simulink model "Inverter_pq_comp"  (R2023b)
settings: Solver=FixedStepDiscrete  StartTime=0.0  StopTime=0.04  RelTol=1e-3  EnableMultiTasking=on
InitFcn:
  | %% Definition of the parameters
  | 
  | Parameter_Definition
  | 
  | %% Damping
  | 
  | Rd = 3.9;
  | 
  | %% PRes Gains Calculation
  | 
  | % Definicao das grandezas
  | w_cl = 1j*2*pi*1200;  % Phase Crossing Frequency
  | no   = 1;           % Integral Resonant Constant
  | A    = 1;             % Carrier Amplitude
  | 
  | % Kp calculation
  | a0 = 1;
  | a1 = Rd*Cf;
  | b0 = 0;
  | b1 = Lf+Lg;
  | b2 = Rd*Lf*Cf+Rd*Lg*Cf;
  | b3 = Lf*Lg*Cf;
  | 
  | G_lcl = (a1*w_cl+a0)/(b3*w_cl^3+b2*w_cl^2+b1*w_cl+b0);
  | % G_lcl = 1/((Lf+Lg)*w_cl+Rf);
  | 
  | G_PWM = (1/A)*(1-w_cl*Ts/4)/(1+w_cl*Ts/4);
  | 
  | G_wc  = (Vdc/2)*(1/I_base)*G_lcl*G_PWM;
  | 
  | G_wc_abs = abs(G_wc);
  | 
  | Kp = 1/G_wc_abs;
  | 
  | % Discretized Controller Gains
  | ressonance_list = [1,5,7];
  | 
  | n_res = length(ressonance_list);
  | a = zeros(2,n_res);
  | b = zeros(2,n_res);
  | Ki_res = zeros(1,n_res);
  | 
  | % for i = 1:n_res
  | %   k = ressonance_list(i);
  | %   Ki_res(i) = (2.2*Kp)/(no*T_gr);
  | %   a(i) = (2*Ki_res(i)*Ts)/(4+((k*w_gr)^2)*Ts^2);
  | %   b(i) = (-8+2*((k*w_gr)^2)*Ts^2)/(4+((k*w_gr)^2)*Ts^2);
  | % end
  | 
  | % wc is the cutoff frequency/damping factor in rad/s
  | wc = 5;
  | 
  | for i = 1:n_res
  |   k = ressonance_list(i);
  |   wk = k * w_gr; % Resonant frequency for this harmonic
  | 
  |   Ki_res(i) = (2.2*Kp)/(0.8*no*T_gr);
  | 
  |   % 1. Calculate the common denominator
  |   den = 4 + 4*wc*Ts + (wk^2)*(Ts^2);
  | ... (+14 lines)
values from neighbouring files (symbols this model uses):
  a1_sogi = single(2*(w0_sogi^2-c_sogi^2)/den0_sogi)    [Parameter_Definition.m]
  a2_sogi = single((c_sogi^2                 - k_sogi*w0_sogi*c_sogi                 + w0_sogi^2)/den0_sogi)    [Parameter_Definition.m]
  bD_sogi = single(k_sogi*w0_sogi*c_sogi/den0_sogi)    [Parameter_Definition.m]
  bQ_sogi = single(k_sogi*w0_sogi^2/den0_sogi)    [Parameter_Definition.m]
  Cf = 5e-6    (= 5e-06)    [Parameter_Definition.m]
  I_base = S_base/(sqrt(3)*V_gr)    [Parameter_Definition.m]
  K_i = 1/25    (= 0.04)    [Parameter_Definition.m]
  K_vc = 1/200    (= 0.005)    [Parameter_Definition.m]
  K_vdc = 1/500    (= 0.002)    [Parameter_Definition.m]
  Lf = 1e-3    (= 0.001)    [Parameter_Definition.m]
  Lg = 0.5e-3    (= 0.0005)    [Parameter_Definition.m]
  S_base = S_rated    (= 1000)    [Parameter_Definition.m]
  Ts = 2*(4167)/100e6    (= 8.334e-05)    [Parameter_Definition.m]
  V_base = sqrt(3)*V_gr    [Parameter_Definition.m]
  Vdc = 800    [Parameter_Definition.m]
  Vdc_base = Vdc    (= 800)    [Parameter_Definition.m]
  w_gr = 2*pi*f_gr    (= 376.991118431)    [Parameter_Definition.m]
undefined symbols (not defined in the file or in its folder): Down, GPTRIP1SEL, TZ1, Up
libraries: c2802xlib x32, c2837xDlib x4, simulink x1
(part 2 of 2)

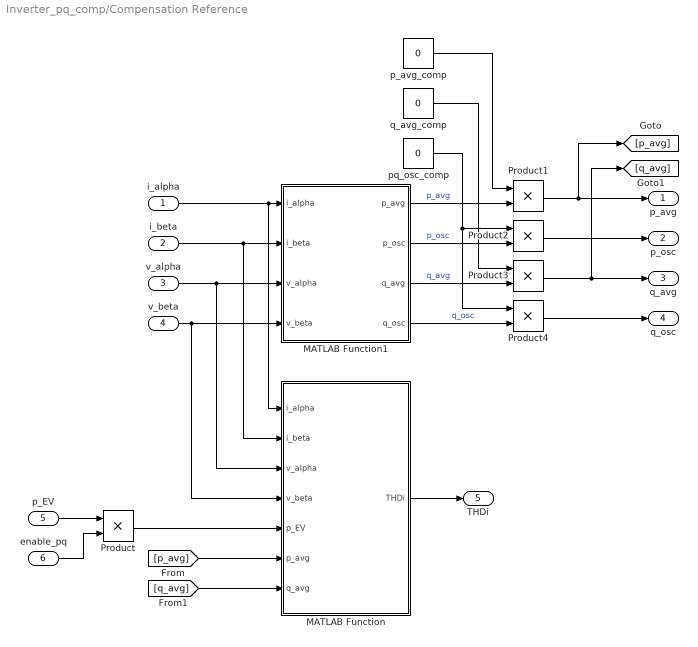
== system Inverter_pq_comp/Compensation Reference ==
  i_alpha : Inport
  i_beta : Inport  Port=2
  v_alpha : Inport  Port=3
  v_beta : Inport  Port=4
  p_EV : Inport  Port=5
  enable_pq : Inport  Port=6
  MATLAB Function : MATLAB Function  TreatAsAtomicUnit=on
  MATLAB Function1 : MATLAB Function  TreatAsAtomicUnit=on
  Product{,1..4} (5 alike) : Product
  p_avg_comp : Constant  Value=0  OutDataTypeStr=single
  pq_osc_comp : Constant  Value=0  OutDataTypeStr=single
  q_avg_comp : Constant  Value=0  OutDataTypeStr=single
  p_avg : Outport
  p_osc : Outport  Port=2
  q_avg : Outport  Port=3
  q_osc : Outport  Port=4
  THDi : Outport  Port=5
  wires:
  MATLAB Function1/1(p_avg) -> Product1/2  "p_avg"
  MATLAB Function1/3(q_avg) -> Product3/2  "q_avg"
  MATLAB Function1/2(p_osc) -> Product2/2  "p_osc"
  i_alpha/1 -> MATLAB Function/1(i_alpha), MATLAB Function1/1(i_alpha)
  MATLAB Function1/4(q_osc) -> Product4/2  "q_osc"
  i_beta/1 -> MATLAB Function/2(i_beta), MATLAB Function1/2(i_beta)
  v_alpha/1 -> MATLAB Function/3(v_alpha), MATLAB Function1/3(v_alpha)
  v_beta/1 -> MATLAB Function/4(v_beta), MATLAB Function1/4(v_beta)
  Product1/1 -> [p_avg], p_avg/1
  Product2/1 -> p_osc/1
  Product3/1 -> [q_avg], q_avg/1
  Product4/1 -> q_osc/1
  [p_avg] -> MATLAB Function/6(p_avg)
  [q_avg] -> MATLAB Function/7(q_avg)
  MATLAB Function/1(THDi) -> THDi/1
  Product/1 -> MATLAB Function/5(p_EV)
  p_EV/1 -> Product/1
  enable_pq/1 -> Product/2
  p_avg_comp/1 -> Product1/1
  q_avg_comp/1 -> Product3/1
  pq_osc_comp/1 -> Product4/1, Product2/1

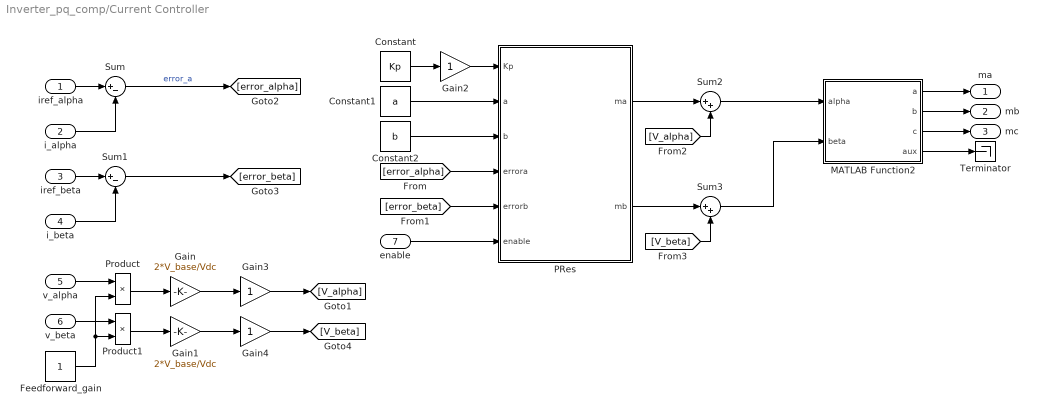
== system Inverter_pq_comp/Current Controller ==
  iref_alpha : Inport
  i_alpha : Inport  Port=2
  iref_beta : Inport  Port=3
  i_beta : Inport  Port=4
  v_alpha : Inport  Port=5
  v_beta : Inport  Port=6
  enable : Inport  Port=7
  Constant : Constant  Value=Kp  OutDataTypeStr=single
  Constant1 : Constant  Value=a  OutDataTypeStr=single
  Constant2 : Constant  Value=b  OutDataTypeStr=single
  Feedforward_gain : Constant  OutDataTypeStr=single
  Gain : Gain  Gain=2*V_base/Vdc
  Gain1 : Gain  Gain=2*V_base/Vdc
  Gain2 : Gain
  Gain3 : Gain
  Gain4 : Gain
  MATLAB Function2 : MATLAB Function  TreatAsAtomicUnit=on
  PRes : MATLAB Function  TreatAsAtomicUnit=on
  Product : Product
  Product1 : Product
  Sum : Sum  Inputs=|+-
  Sum1 : Sum  Inputs=|+-
  Sum2 : Sum  Inputs=|++
  Sum3 : Sum  Inputs=|++
  Terminator : Terminator
  ma : Outport
  mb : Outport  Port=2
  mc : Outport  Port=3
  wires:
  Constant1/1 -> PRes/2(a)
  Constant2/1 -> PRes/3(b)
  [error_alpha] -> PRes/4(errora)
  [error_beta] -> PRes/5(errorb)
  iref_alpha/1 -> Sum/1
  i_alpha/1 -> Sum/2
  iref_beta/1 -> Sum1/1
  i_beta/1 -> Sum1/2
  Sum1/1 -> [error_beta]
  Sum/1 -> [error_alpha]  "error_a"
  enable/1 -> PRes/6(enable)
  PRes/1(ma) -> Sum2/1
  Sum2/1 -> MATLAB Function2/1(alpha)
  PRes/2(mb) -> Sum3/1
  [V_alpha] -> Sum2/2
  [V_beta] -> Sum3/2
  v_beta/1 -> Product1/1
  Product1/1 -> Gain1/1
  v_alpha/1 -> Product/1
  Product/1 -> Gain/1
  Feedforward_gain/1 -> Product/2, Product1/2
  Constant/1 -> Gain2/1
  MATLAB Function2/1(a) -> ma/1
  MATLAB Function2/2(b) -> mb/1
  MATLAB Function2/3(c) -> mc/1
  MATLAB Function2/4(aux) -> Terminator/1
  Sum3/1 -> MATLAB Function2/2(beta)
  Gain/1 -> Gain3/1
  Gain1/1 -> Gain4/1
  Gain2/1 -> PRes/1(Kp)
  Gain3/1 -> [V_alpha]
  Gain4/1 -> [V_beta]

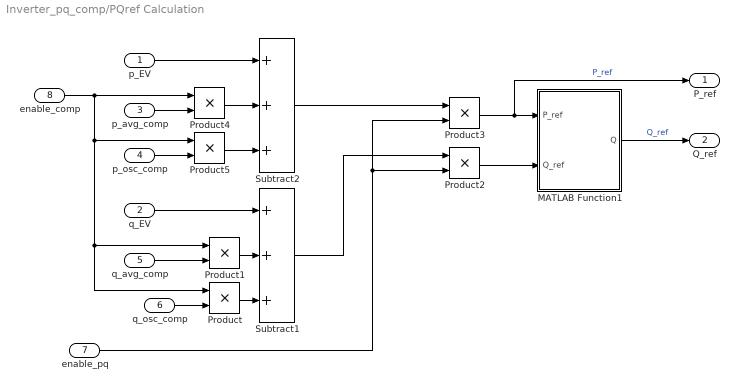
== system Inverter_pq_comp/PQref Calculation ==
  p_EV : Inport
  q_EV : Inport  Port=2
  p_avg_comp : Inport  Port=3
  p_osc_comp : Inport  Port=4
  q_avg_comp : Inport  Port=5
  q_osc_comp : Inport  Port=6
  enable_pq : Inport  Port=7
  enable_comp : Inport  Port=8
  MATLAB Function1 : MATLAB Function  TreatAsAtomicUnit=on
  Product{,1..5} (6 alike) : Product
  Subtract1 : Sum  Inputs=+++
  Subtract2 : Sum  Inputs=+++
  P_ref : Outport
  Q_ref : Outport  Port=2
  wires:
  p_osc_comp/1 -> Product5/2
  Product/1 -> Subtract1/3
  MATLAB Function1/1(Q) -> Q_ref/1  "Q_ref"
  Product1/1 -> Subtract1/2
  p_avg_comp/1 -> Product4/2
  q_osc_comp/1 -> Product/2
  q_avg_comp/1 -> Product1/2
  Product4/1 -> Subtract2/2
  p_EV/1 -> Subtract2/1
  Product5/1 -> Subtract2/3
  q_EV/1 -> Subtract1/1
  Subtract1/1 -> Product2/1
  Product2/1 -> MATLAB Function1/2(Q_ref)
  Product3/1 -> P_ref/1, MATLAB Function1/1(P_ref)  "P_ref"
  enable_pq/1 -> Product3/2, Product2/2
  Subtract2/1 -> Product3/1
  enable_comp/1 -> Product/1, Product1/1, Product5/1, Product4/1

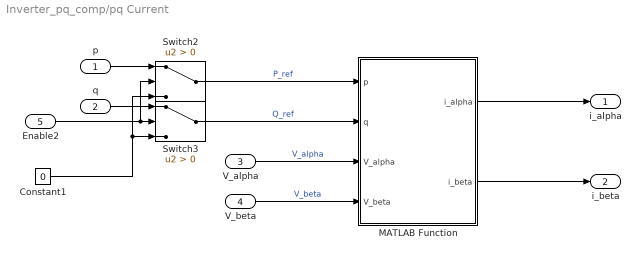
== system Inverter_pq_comp/pq Current ==
  p : Inport
  q : Inport  Port=2
  V_alpha : Inport  Port=3
  V_beta : Inport  Port=4
  Enable2 : Inport  Port=5
  Constant1 : Constant  Value=0  OutDataTypeStr=single
  MATLAB Function : MATLAB Function  TreatAsAtomicUnit=on
  Switch2 : Switch  Criteria=u2 > Threshold  SaturateOnIntegerOverflow=off  InputSameDT=off
  Switch3 : Switch  Criteria=u2 > Threshold  SaturateOnIntegerOverflow=off  InputSameDT=off
  i_alpha : Outport
  i_beta : Outport  Port=2
  wires:
  V_beta/1 -> MATLAB Function/4(V_beta)  "V_beta"
  V_alpha/1 -> MATLAB Function/3(V_alpha)  "V_alpha"
  MATLAB Function/1(i_alpha) -> i_alpha/1
  MATLAB Function/2(i_beta) -> i_beta/1
  p/1 -> Switch2/1
  Switch3/1 -> MATLAB Function/2(q)  "Q_ref"
  q/1 -> Switch3/1
  Constant1/1 -> Switch2/3, Switch3/3
  Enable2/1 -> Switch2/2, Switch3/2
  Switch2/1 -> MATLAB Function/1(p)  "P_ref"

== matlab function Inverter_pq_comp/RMS_fcn4 ==
  data: RMSin input; yout output
function yout = fcn(RMSin)

win = 200;

persistent sampleRMS
    if isempty(sampleRMS)
        sampleRMS = single(0.0);
    end
    if sampleRMS>=win
        sampleRMS = single(0.0);
    end

persistent RMSout
if isempty(RMSout)
    RMSout = single(0.0);
end    
persistent sumRMS
if isempty(sumRMS)
    sumRMS = single(0.0);
end
persistent RMSinArray
     if isempty(RMSinArray)
         RMSinArray = zeros(1,win);
     end

sampleRMS = sampleRMS + 1;      

%RMS of Input Signal
sumRMS = sumRMS + RMSin*RMSin - RMSinArray(1,sampleRMS);
RMSinArray(1,sampleRMS) = RMSin*RMSin;
if sumRMS>=0.0
    RMSout = sqrt(sumRMS/win);
end

%RMSout = RMSout_temp;

yout = RMSout;

== matlab function Inverter_pq_comp/RMS_fcn5 ==
  data: RMSin input; yout output
function yout = fcn(RMSin)

win = 200;

persistent sampleRMS
    if isempty(sampleRMS)
        sampleRMS = single(0.0);
    end
    if sampleRMS>=win
        sampleRMS = single(0.0);
    end

persistent RMSout
if isempty(RMSout)
    RMSout = single(0.0);
end    
persistent sumRMS
if isempty(sumRMS)
    sumRMS = single(0.0);
end
persistent RMSinArray
     if isempty(RMSinArray)
         RMSinArray = zeros(1,win);
     end

sampleRMS = sampleRMS + 1;      

%RMS of Input Signal
sumRMS = sumRMS + RMSin*RMSin - RMSinArray(1,sampleRMS);
RMSinArray(1,sampleRMS) = RMSin*RMSin;
if sumRMS>=0.0
    RMSout = sqrt(sumRMS/win);
end

%RMSout = RMSout_temp;

yout = RMSout;

== matlab function Inverter_pq_comp/Compensation Reference/MATLAB Function1 ==
  data: i_alpha input; p_avg output; i_beta input; v_alpha input; v_beta input; p_osc output; q_avg output; q_osc output
function [p_avg, p_osc, q_avg, q_osc] = pqCalc(i_alpha, i_beta, v_alpha, v_beta)
    % Initial logic and parameters are validated. 
    % Standard processing applied for spatial vector alignment.

    persistent buffer_p buffer_q sum_p sum_q idx
    window = 200; % Must match your 12000Hz/60Hz window size exactly
    
    if isempty(buffer_p)
        buffer_p = zeros(window, 1);
        buffer_q = zeros(window, 1);
        sum_p = single(0.0);
        sum_q = single(0.0);
        idx = 1;
    end
    
    % Final transformation: Strip scaling coefficients to match I_total_sq domain
    p = (v_alpha * i_alpha) + (v_beta * i_beta);
    q = (v_beta * i_alpha) - (v_alpha * i_beta);
    
    % Align filter topology to match current/voltage sliding window
    old_p = buffer_p(idx);
    old_q = buffer_q(idx);
    
    buffer_p(idx) = p;
    buffer_q(idx) = q;
    
    sum_p = sum_p + p - old_p;
    sum_q = sum_q + q - old_q;
    
    idx = idx + 1;
    if idx > window
        idx = 1;
    end
    
    p_avg = sum_p / window;
    q_avg = sum_q / window;
    
    p_osc = p - p_avg;
    q_osc = q - q_avg;
end

== matlab function Inverter_pq_comp/MATLAB Function11 ==
  data: i_rms input; error_overcurrent output; error_ac_overvoltage output; error_dc_overvoltage output; error_unbalance output; error_low_Vdc output; enable_contactor_out output; enable_PreCharge_out output; enable_PWM_out output; enable_PQ_out output; enable_comp_out output; enable_Feedforward_out output; I_limit input; V_rms input; V_limit input; V_dc input; Vdc_limit input; V_unb input; Vunb_limit input; enable_relay input; enable_PWM input; enable_PreCharge input; enable_PQ input; enable_comp input; error_reset input; error_reset_out output; out_gpio output
function [error_overcurrent, error_ac_overvoltage, error_dc_overvoltage, error_unbalance, error_low_Vdc, enable_contactor_out, enable_PreCharge_out, enable_PWM_out, enable_PQ_out, enable_comp_out, enable_Feedforward_out, error_reset_out, out_gpio] = TNPC_Protection(i_rms, I_limit, V_rms, V_limit, V_dc, Vdc_limit, V_unb, Vunb_limit, enable_relay, enable_PWM, enable_PreCharge, enable_PQ, enable_comp, error_reset)

% Persistent variables definition
persistent error_flag
persistent error_overcurrent_p
persistent error_ac_overvoltage_p
persistent error_dc_overvoltage_p
persistent error_unbalance_p
persistent error_low_Vdc_p
persistent count_I_limit
if isempty(error_flag)
    error_flag = single(0);
    error_overcurrent_p    = single(0);
    error_ac_overvoltage_p = single(0);
    error_dc_overvoltage_p = single(0);
    error_unbalance_p      = single(0);
    error_low_Vdc_p        = single(0);
    count_I_limit          = int16(0);
end


out_Feedforward = single(0.0);
% Count to keep high current limit in first 15 cycles
if enable_relay == 1
    if count_I_limit < 10*200
        I_limit = single(100.0);
        count_I_limit = count_I_limit + 1;
        out_Feedforward = single(1.0);
    elseif count_I_limit < 15*200
        I_limit = single(100.0);
        count_I_limit = count_I_limit + 1;
        out_Feedforward = single(0.0);
    end
end

enable_Feedforward_out = out_Feedforward;

% Check for errors
if max(i_rms) > I_limit
    error_overcurrent = single(1);
    error_overcurrent_p = single(1);
else
    error_overcurrent = single(0);
end

if V_dc > Vdc_limit
    error_dc_overvoltage = single(1);
    error_dc_overvoltage_p = single(1);
else
    error_dc_overvoltage = single(0);  
end

if V_unb > Vunb_limit
    error_unbalance = single(1);
    error_unbalance_p = single(1);
else
    error_unbalance = single(0);
end

if max(V_rms) > V_limit
    error_ac_overvoltage = single(1);
    error_ac_overvoltage_p = single(1);
else
    error_ac_overvoltage = single(0);  
end

if V_dc*500 < sqrt(2)*max(V_rms)*250
    error_low_Vdc = single(1);
    error_low_Vdc_p = single(1);
else
    error_low_Vdc = single(0);
end

% Raise the error flag
if (error_overcurrent == 1) || (error_dc_overvoltage == 1) || (error_unbalance == 1) || (error_ac_overvoltage == 1) || (error_low_Vdc == 1)
    error_flag = single(1);
end

% Reset logic
if error_flag == 1 && error_reset == 1 && error_overcurrent == 0 && error_dc_overvoltage == 0 && error_ac_overvoltage == 0 && error_unbalance == 0 && error_low_Vdc == 0
    % Clear the persistent variables
    error_flag = single(0);
    error_overcurrent_p    = single(0);
    error_ac_overvoltage_p = single(0);
    error_dc_overvoltage_p = single(0);
    error_unbalance_p      = single(0);
    error_low_Vdc_p        = single(0);
    count_I_limit          = int16(0);
    % Send 0 to the reset signal
    error_reset_out = single(0);
else
    error_reset_out = error_reset;
end

% Enable signals output
if error_flag == 1
    enable_contactor_out = single(0);
    enable_PWM_out       = single(0);
    enable_PreCharge_out = single(0);
    enable_PQ_out        = single(0);
    enable_comp_out      = single(0);
else
    enable_contactor_out = enable_relay;
    enable_PWM_out       = enable_PWM;
    enable_PreCharge_out = enable_PreCharge;
    enable_PQ_out        = enable_PQ;
    enable_comp_out      = enable_comp;
end

if (error_overcurrent_p == 1) || (error_dc_overvoltage_p == 1) || (error_unbalance_p == 1) || (error_ac_overvoltage_p == 1) || (error_low_Vdc_p == 1)
    out_gpio = single(1);
else
    out_gpio = single(0);
end

== matlab function Inverter_pq_comp/PQref Calculation/MATLAB Function1 ==
  data: P_ref input; Q_ref input; Q output
function Q = Q_limit(P_ref, Q_ref)

Smax = single(1.0);

if P_ref > 1
    P_ref = single(1.0);
end

Qmax = sqrt(Smax^2-P_ref^2);

if Qmax > abs(Q_ref)
    Q = Q_ref;
else
    Q = Qmax*sign(Q_ref);
end

== matlab function Inverter_pq_comp/Current Controller/PRes ==
  data: Kp input; a input; b input; errora input; ma output; errorb input; mb output; enable input
function [ma, mb] = PResCurrent(Kp, a, b, errora, errorb, enable)

%Controller modeled in abc frame, considering p.u. values

%%% Variables Definition
%%%%#########################################################
%%%%######################################################### 

nRes = length(a);

max_pu = single(1.0);

%Proportional part variable
%Phase a
persistent pia
    if isempty(pia)
        pia = single(0.0);
    end
%Phase b    
persistent pib
    if isempty(pib)
        pib = single(0.0);
    end 
    
%Resonant parts variables
%Phase a
persistent presa
    if isempty(presa)
        presa = zeros(1,nRes);
    end
persistent presa_1d %1 sample delay
    if isempty(presa_1d)
        presa_1d = zeros(1,nRes);
    end    
persistent presa_2d %2 samples delay
    if isempty(presa_2d)
        presa_2d = zeros(1,nRes);
    end
persistent presOUT_ia
    if isempty(presOUT_ia)
        presOUT_ia = single(0.0);
    end
    
%Phase b
persistent presb
    if isempty(presb)
        presb = zeros(1,nRes);
    end
persistent presb_1d %1 sample delay
    if isempty(presb_1d)
        presb_1d = zeros(1,nRes);
    end    
persistent presb_2d %2 samples delay
    if isempty(presb_2d)
        presb_2d = zeros(1,nRes);
    end
persistent presOUT_ib
    if isempty(presOUT_ib)
        presOUT_ib = single(0.0);
    end

%Error variables
%Phase a
% persistent errora %Actual error
%     if isempty(errora)
%         errora = 0.0;
%     end
persistent errora_0d %Actual error to delay
    if isempty(errora_0d)
        errora_0d = single(0.0);
    end
persistent errora_1d %1 sample delay
    if isempty(errora_1d)
        errora_1d = single(0.0);
    end    
persistent errora_2d %2 sample delay
    if isempty(errora_2d)
        errora_2d = single(0.0);
    end   
%Phase b
% persistent errorb %Actual error
%     if isempty(errorb)
%         errorb = 0.0;
%     end
persistent errorb_0d %Actual error to delay
    if isempty(errorb_0d)
        errorb_0d = single(0.0);
    end
persistent errorb_1d %1 sample delay
    if isempty(errorb_1d)
        errorb_1d = single(0.0);
    end    
persistent errorb_2d %2 sample delay
    if isempty(errorb_2d)
        errorb_2d = single(0.0);
    end

%%% Enable logic
%%%%#########################################################
%%%%#########################################################

if ~enable 
    % Define safe outputs
    ma = single(0.0);
    mb = single(0.0);
    mc = single(0.0);
    
    % Reset history registers for bumpless transfer
    pia = single(0.0); pib = single(0.0);
    
    presa       = zeros(1,nRes);
    presa_1d    = zeros(1,nRes);
    presa_2d    = zeros(1,nRes);
    presOUT_ia  = single(0.0);
    
    presb       = zeros(1,nRes);
    presb_1d    = zeros(1,nRes);
    presb_2d    = zeros(1,nRes);
    presOUT_ib  = single(0.0);
    
    errora_0d = single(0.0); errora_1d = single(0.0); errora_2d = single(0.0);
    errorb_0d = single(0.0); errorb_1d = single(0.0); errorb_2d = single(0.0);
    
    % Exit the function completely
    return; 
end

%%% PRes Current Controllers
%%%%#########################################################
%%%%#########################################################

%Proportional part
pia = errora*Kp;
pib = errorb*Kp;
    
    %Saturation - a
    if pia > max_pu 
        pia = max_pu;
    end
    if pia < -1*max_pu
        pia = -1*max_pu;
    end
    %Saturation - b
    if pib > max_pu
        pib = max_pu;
    end
    if pib < -1*max_pu
        pib = -1*max_pu;
    end   
    
    % %Anti-windup - a
    % if pia > 0.0
    %     limit_ia = max_pu - pia;
    % else
    %     limit_ia = 1 + pia;
    % end
    %  %Anti-windup - b
    % if pib > 0.0
    %     limit_ib = max_pu - pib;
    % else
    %     limit_ib = 1 + pib;
    % end
%     %Anti-windup - c
%     if pic > 0.0
%         limit_ic = max_pu - pic;
%     else
%         limit_ic = 1 + pic;
%     end    
    
    
%Resonant part
errora_2d = errora_1d;
errora_1d = errora_0d;
errora_0d = errora;

errorb_2d = errorb_1d;
errorb_1d = errorb_0d;
errorb_0d = errorb;
        
for i=1:nRes

    %leg a
    presa_2d(i) = presa_1d(i);
	presa_1d(i) = presa(i);
	presa(i) = a(1,i)*errora + a(2,i)*errora_2d - b(1,i)*presa_1d(i) - b(2,i)*presa_2d(i);    
    % if presa(i) > limit_ia
    %     presa(i) = limit_ia;
    % end
    % if presa(i) < -1*limit_ia
    %     presa(i) = -1*limit_ia;
    % end
 
    %leg b
    presb_2d(i) = presb_1d(i);
	presb_1d(i) = presb(i);
	presb(i) = a(1,i)*errorb + a(2,i)*errorb_2d - b(1,i)*presb_1d(i) - b(2,i)*presb_2d(i);    
    % if presb(i) > limit_ib
    %     presb(i) = limit_ib;
    % end
    % if presb(i) < -1*limit_ib
    %     presb(i) = -1*limit_ib;
    % end  
    
end

presOUT_ia = pia;
presOUT_ib = pib;

for i=1:nRes
    presOUT_ia = presOUT_ia + presa(i);
    presOUT_ib = presOUT_ib + presb(i);  
end

%Output for PWM
ma = presOUT_ia;
        %Saturation - ta
        if ma > max_pu 
            ma = max_pu;
        end
        if ma < -1*max_pu
            ma = -1*max_pu;
        end

mb = presOUT_ib;
        %Saturation - tb
        if mb > max_pu 
            mb = max_pu;
        end
        if mb < -1*max_pu
            mb = -1*max_pu;
        end
        
end

== matlab function Inverter_pq_comp/Current Controller/MATLAB Function2 ==
  data: alpha input; a output; beta input; b output; c output; aux output
function [a, b, c, aux] = abc(alpha, beta)

a = sqrt(2/3)*alpha;
b = sqrt(2/3)*(-1*alpha/2 + sqrt(3)*beta/2);
c = sqrt(2/3)*(-1*alpha/2 - sqrt(3)*beta/2);

max_mod = max(abs([a, b, c]));

if max_mod > 1
    scale = 1/max_mod;

    a = a*scale;
    b = b*scale;
    c = c*scale;

    aux = single(1.0);
else
    aux = single(0.0);
end

== matlab function Inverter_pq_comp/MATLAB Function3 ==
  data: a input; alpha output; b input; c input; beta output
function [alpha, beta] = alpha_beta(a, b, c)

alpha = sqrt(2/3)*(a - b/2 - c/2);
beta  = sqrt(2/3)*(sqrt(3)*b/2 - sqrt(3)*c/2);

== matlab function Inverter_pq_comp/pq Current/MATLAB Function ==
  data: p input; i_alpha output; q input; i_beta output; V_alpha input; V_beta input
function [i_alpha, i_beta] = pq_to_i(p, q, V_alpha, V_beta)

i_alpha = (1/(V_alpha^2+V_beta^2))*(V_alpha*p + V_beta*q);
i_beta  = (1/(V_alpha^2+V_beta^2))*(V_beta*p - V_alpha*q);

== matlab function Inverter_pq_comp/Compensation Reference/MATLAB Function ==
  data: i_alpha input; THDi output; i_beta input; v_alpha input; v_beta input; p_EV input; p_avg input; q_avg input
function THDi = THD_calc( ...
    i_alpha, i_beta, ...
    v_alpha, v_beta, ...
    p_EV, p_avg, q_avg)
%#codegen

    window = 200;
    epsilon = 1e-9;

    persistent buffer_I_total;
    persistent buffer_V;
    persistent sum_I_total;
    persistent sum_V;
    persistent idx;
    persistent count;

    if isempty(idx)
        buffer_I_total = zeros(window,1);
        buffer_V = zeros(window,1);

        sum_I_total = single(0.0);
        sum_V = single(0.0);

        idx = 1;
        count = 0;
    end

    % Load-current magnitude squared
    I_total_inst_sq = i_alpha^2 + i_beta^2;

    % Fundamental PCC-voltage magnitude squared
    V_inst_sq = v_alpha^2 + v_beta^2;

    % Remove oldest samples
    old_I = buffer_I_total(idx);
    old_V = buffer_V(idx);

    % Insert newest samples
    buffer_I_total(idx) = I_total_inst_sq;
    buffer_V(idx) = V_inst_sq;

    % Update moving sums
    sum_I_total = ...
        sum_I_total + I_total_inst_sq - old_I;

    sum_V = ...
        sum_V + V_inst_sq - old_V;

    idx = idx + 1;

    if idx > window
        idx = 1;
    end

    if count < window
        count = count + 1;
    end

    % Do not calculate THD before one complete cycle
    if count < window
        THDi = single(0.0);
        return;
    end

    % Squared total load-current magnitude
    IL_total_sq = max(sum_I_total/window,0);

    % Squared fundamental voltage magnitude
    V1_sq = max(sum_V/window,epsilon);

    % Fundamental LOAD current
    IL_fund_sq = ...
        (p_avg^2 + q_avg^2)/V1_sq;

    % Harmonic LOAD current
    IH_load_sq = max( ...
        IL_total_sq - IL_fund_sq, ...
        0);

    % Fundamental grid current including EV charging
    %
    % Current convention:
    % p_EV is negative during charging.
    p_total_fund = p_avg - p_EV;

    IT_fund_sq = ...
        (p_total_fund^2 + q_avg^2)/V1_sq;

    % Equivalent pre-compensation grid THD
    if IT_fund_sq <= epsilon
        THDi = single(0.0);
    else
        THDi = sqrt(IH_load_sq/IT_fund_sq);
    end
end

== matlab function Inverter_pq_comp/MATLAB Function1 ==
  data: a input; alpha output; b input; c input; beta output
function [alpha, beta] = alpha_beta(a, b, c)

alpha = sqrt(2/3)*(a - b/2 - c/2);
beta  = sqrt(2/3)*(sqrt(3)*b/2 - sqrt(3)*c/2);

== matlab function Inverter_pq_comp/MATLAB Function ==
  data: v_unf input; v_f output; bD input; bQ input; a1 input; a2 input; enable input
function v_f  = SOGI(v_unf, bD, bQ, a1, a2, enable)

persistent u1 u2
persistent vf1 vf2
persistent vq1 vq2

if isempty(u1)
    u1  = single(0);
    u2  = single(0);

    vf1 = single(0);
    vf2 = single(0);

    vq1 = single(0);
    vq2 = single(0);
end

if enable == 0
    u1  = single(0);
    u2  = single(0);

    vf1 = single(0);
    vf2 = single(0);

    vq1 = single(0);
    vq2 = single(0);

    v_f = single(0);
    v_q = single(0);
    return;
end

u   = single(v_unf);
bd  = single(bD);
bq  = single(bQ);
aa1 = single(a1);
aa2 = single(a2);

% In-phase band-pass output
v_f = bd*(u - u2) ...
    - aa1*vf1 ...
    - aa2*vf2;

% Quadrature output
v_q = bq*(u + single(2)*u1 + u2) ...
    - aa1*vq1 ...
    - aa2*vq2;

% Update histories AFTER calculating both outputs
u2 = u1;
u1 = u;

vf2 = vf1;
vf1 = v_f;

vq2 = vq1;
vq1 = v_q;

end

== matlab function Inverter_pq_comp/MATLAB Function4 ==
  data: v_unf input; v_f output; bD input; bQ input; a1 input; a2 input; enable input
function v_f  = SOGI(v_unf, bD, bQ, a1, a2, enable)

persistent u1 u2
persistent vf1 vf2
persistent vq1 vq2

if isempty(u1)
    u1  = single(0);
    u2  = single(0);

    vf1 = single(0);
    vf2 = single(0);

    vq1 = single(0);
    vq2 = single(0);
end

if enable == 0
    u1  = single(0);
    u2  = single(0);

    vf1 = single(0);
    vf2 = single(0);

    vq1 = single(0);
    vq2 = single(0);

    v_f = single(0);
    v_q = single(0);
    return;
end

u   = single(v_unf);
bd  = single(bD);
bq  = single(bQ);
aa1 = single(a1);
aa2 = single(a2);

% In-phase band-pass output
v_f = bd*(u - u2) ...
    - aa1*vf1 ...
    - aa2*vf2;

% Quadrature output
v_q = bq*(u + single(2)*u1 + u2) ...
    - aa1*vq1 ...
    - aa2*vq2;

% Update histories AFTER calculating both outputs
u2 = u1;
u1 = u;

vf2 = vf1;
vf1 = v_f;

vq2 = vq1;
vq1 = v_q;

end

== matlab function Inverter_pq_comp/MATLAB Function2 ==
  data: a input; alpha output; b input; c input; beta output
function [alpha, beta] = alpha_beta(a, b, c)

alpha = sqrt(2/3)*(a - b/2 - c/2);
beta  = sqrt(2/3)*(sqrt(3)*b/2 - sqrt(3)*c/2);

== matlab function Inverter_pq_comp/RMS_fcn ==
  data: RMSin input; yout output
function yout = fcn(RMSin)

win = 200;

persistent sampleRMS
    if isempty(sampleRMS)
        sampleRMS = single(0.0);
    end
    if sampleRMS>=win
        sampleRMS = single(0.0);
    end

persistent RMSout
if isempty(RMSout)
    RMSout = single(0.0);
end    
persistent sumRMS
if isempty(sumRMS)
    sumRMS = single(0.0);
end
persistent RMSinArray
     if isempty(RMSinArray)
         RMSinArray = zeros(1,win);
     end

sampleRMS = sampleRMS + 1;      

%RMS of Input Signal
sumRMS = sumRMS + RMSin*RMSin - RMSinArray(1,sampleRMS);
RMSinArray(1,sampleRMS) = RMSin*RMSin;
if sumRMS>=0.0
    RMSout = sqrt(sumRMS/win);
end

%RMSout = RMSout_temp;

yout = RMSout;

== matlab function Inverter_pq_comp/RMS_fcn1 ==
  data: RMSin input; yout output
function yout = fcn(RMSin)

win = 200;

persistent sampleRMS
    if isempty(sampleRMS)
        sampleRMS = single(0.0);
    end
    if sampleRMS>=win
        sampleRMS = single(0.0);
    end

persistent RMSout
if isempty(RMSout)
    RMSout = single(0.0);
end    
persistent sumRMS
if isempty(sumRMS)
    sumRMS = single(0.0);
end
persistent RMSinArray
     if isempty(RMSinArray)
         RMSinArray = zeros(1,win);
     end

sampleRMS = sampleRMS + 1;      

%RMS of Input Signal
sumRMS = sumRMS + RMSin*RMSin - RMSinArray(1,sampleRMS);
RMSinArray(1,sampleRMS) = RMSin*RMSin;
if sumRMS>=0.0
    RMSout = sqrt(sumRMS/win);
end

%RMSout = RMSout_temp;

yout = RMSout;

== matlab function Inverter_pq_comp/RMS_fcn2 ==
  data: RMSin input; yout output
function yout = fcn(RMSin)

win = 200;

persistent sampleRMS
    if isempty(sampleRMS)
        sampleRMS = single(0.0);
    end
    if sampleRMS>=win
        sampleRMS = single(0.0);
    end

persistent RMSout
if isempty(RMSout)
    RMSout = single(0.0);
end    
persistent sumRMS
if isempty(sumRMS)
    sumRMS = single(0.0);
end
persistent RMSinArray
     if isempty(RMSinArray)
         RMSinArray = zeros(1,win);
     end

sampleRMS = sampleRMS + 1;      

%RMS of Input Signal
sumRMS = sumRMS + RMSin*RMSin - RMSinArray(1,sampleRMS);
RMSinArray(1,sampleRMS) = RMSin*RMSin;
if sumRMS>=0.0
    RMSout = sqrt(sumRMS/win);
end

%RMSout = RMSout_temp;

yout = RMSout;

== matlab function Inverter_pq_comp/RMS_fcn3 ==
  data: RMSin input; yout output
function yout = fcn(RMSin)

win = 200;

persistent sampleRMS
    if isempty(sampleRMS)
        sampleRMS = single(0.0);
    end
    if sampleRMS>=win
        sampleRMS = single(0.0);
    end

persistent RMSout
if isempty(RMSout)
    RMSout = single(0.0);
end    
persistent sumRMS
if isempty(sumRMS)
    sumRMS = single(0.0);
end
persistent RMSinArray
     if isempty(RMSinArray)
         RMSinArray = zeros(1,win);
     end

sampleRMS = sampleRMS + 1;      

%RMS of Input Signal
sumRMS = sumRMS + RMSin*RMSin - RMSinArray(1,sampleRMS);
RMSinArray(1,sampleRMS) = RMSin*RMSin;
if sumRMS>=0.0
    RMSout = sqrt(sumRMS/win);
end

%RMSout = RMSout_temp;

yout = RMSout;
